simulink model "BMS_OV_Protection_Test"  (R2025b)
settings: Solver=FixedStepDiscrete  StartTime=0.0  StopTime=6  FixedStep=Ts  RelTol=1e-3
undefined symbols (not defined in the file): Ts
settings Model: Creator=Khadija  LastModifiedBy=Khadija

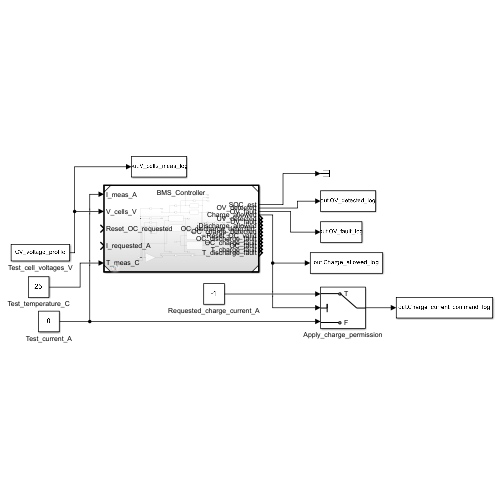
[thumbnail: Simulink's stored preview of the top-level diagram]
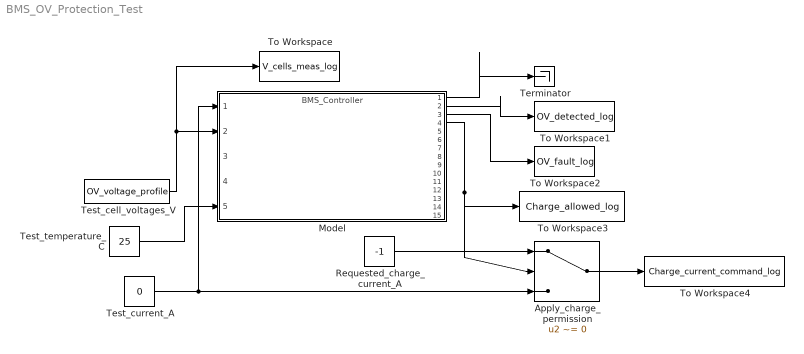
== system BMS_OV_Protection_Test ==
  Apply_charge_permission : Switch  Criteria=u2 ~= 0  SaturateOnIntegerOverflow=off  InputSameDT=off
  Model : ModelReference  ModelNameDialog=BMS_Controller  SimulationMode=Normal  ModelReferenceVersion=1.40
  Requested_charge_current_A : Constant  Value=-1  SampleTime=Ts
  Terminator : Terminator
  Test_cell_voltages_V : FromWorkspace  VariableName=OV_voltage_profile  SampleTime=Ts  Interpolate=off  ZeroCross=off  OutputAfterFinalValue=Holding final value
  Test_current_A : Constant  Value=0  SampleTime=Ts
  Test_temperature_C : Constant  Value=25  OutDataTypeStr=double  SampleTime=Ts
  To Workspace : ToWorkspace  VariableName=V_cells_meas_log  SaveFormat=Timeseries  SampleTime=-1
  To Workspace1 : ToWorkspace  VariableName=OV_detected_log  SaveFormat=Timeseries  SampleTime=-1
  To Workspace2 : ToWorkspace  VariableName=OV_fault_log  SaveFormat=Timeseries  SampleTime=-1
  To Workspace3 : ToWorkspace  VariableName=Charge_allowed_log  SaveFormat=Timeseries  SampleTime=-1
  To Workspace4 : ToWorkspace  VariableName=Charge_current_command_log  SaveFormat=Timeseries  SampleTime=-1
  wires:
  Model/4 -> Apply_charge_permission/2, To Workspace3/1
  Model/3 -> To Workspace2/1
  Model/2 -> To Workspace1/1
  Test_current_A/1 -> Apply_charge_permission/3, Model/1
  Test_cell_voltages_V/1 -> To Workspace/1, Model/2
  Apply_charge_permission/1 -> To Workspace4/1
  Model/1 -> Terminator/1
  Requested_charge_current_A/1 -> Apply_charge_permission/1
  Test_temperature_C/1 -> Model/5
